simulink model "First"  (R2025b)
settings: Solver=VariableStepAuto  StartTime=0.0  StopTime=10.0  RelTol=1e-3
settings Model: Creator=samue  LastModifiedBy=samue

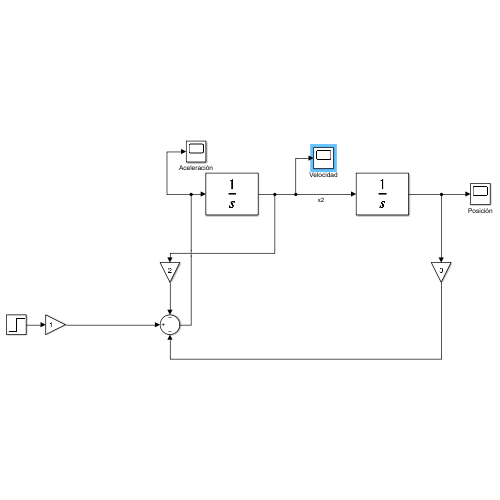
[thumbnail: Simulink's stored preview of the top-level diagram]
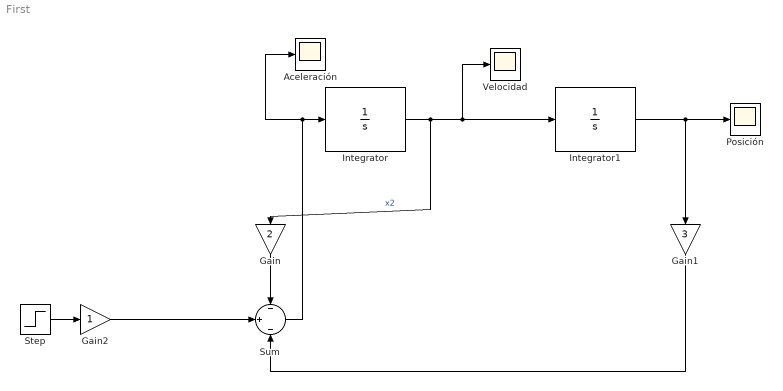
== system First ==
  Aceleración : Scope
      settings: ActiveDisplayYMinimum=-2278.5031534180439  ActiveDisplayYMaximum=506.52838076239561  DataLoggingVariableName=ScopeData2
  Gain : Gain  Gain=2
  Gain1 : Gain  Gain=3
  Gain2 : Gain
  Integrator : Integrator  InitialCondition=1000
  Integrator1 : Integrator
  Posición : Scope
      settings: ActiveDisplayYMinimum=-72.0144243624344  ActiveDisplayYMaximum=334.21292833145804
  Step : Step  After=0  SampleTime=0
  Sum : Sum  Inputs=-|+|-
  Velocidad : Scope
      settings: ActiveDisplayYMinimum=-415.33339479913616  ActiveDisplayYMaximum=1157.2592660887929
  wires:
  Integrator/1 -> Velocidad/1, Integrator1/1, Gain/1  "x2"
  Integrator1/1 -> Posición/1, Gain1/1
  Step/1 -> Gain2/1
  Gain1/1 -> Sum/3
  Sum/1 -> Aceleración/1, Integrator/1
  Gain/1 -> Sum/1
  Gain2/1 -> Sum/2
